simulink model "Fourteen_bus_simscape_V1o1"  (R2026a)
settings: Solver=ode23t  StopTime=12  FixedStep=0.2  RelTol=1e-2  AbsTol=1e-2  EnableMultiTasking=on
libraries: ee_lib x92, nesl_utility x64, fl_lib x25, eeRmsMeasurement x18, slpidlib x5, eeSmGovernor x2, elec_conv_HighZElecRef x1
(part 3 of 3)

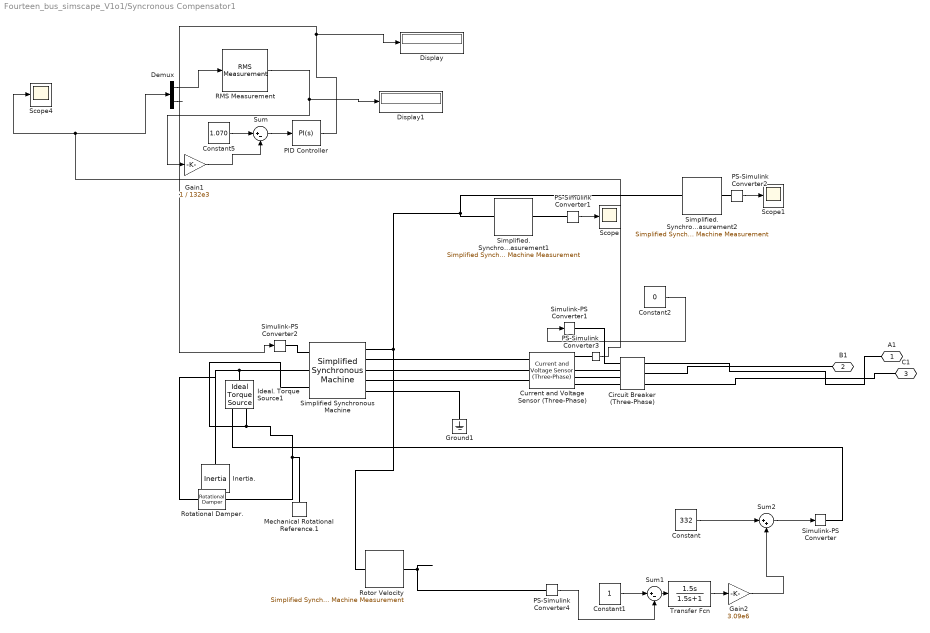
== system Fourteen_bus_simscape_V1o1/Syncronous Compensator1 ==
  Circuit Breaker (Three-Phase) : ee_lib/Switches & Breakers/Circuit Breaker (Three-Phase)  port_option=ee.enum.threePhasePort.expanded  control_port_option=ee.enum.controlport.ps  R_closed=0.001 Ohm  G_open=1e-6 1/Ohm  threshold=0.5 V  breaker_behavior=ee.enum.switches.breakerBehavior.zeroCrossingDisable  i_th=1e-8 A
  Constant : Constant  Value=332
  Constant1 : Constant
  Constant2 : Constant  Value=0
  Constant5 : Constant  Value=1.070
  Current and Voltage Sensor (Three-Phase) : ee_lib/Sensors & Transducers/Current and Voltage Sensor (Three-Phase)  port_option=ee.enum.threePhasePort.expanded  vMeasurementType=ee.enum.vmeasurement.ll  outputUnit=ee.enum.unit.si  SRated=100000000 V*A  VRated=0.95 V  I_specify=off  I_priority=None  I=[ 0 0 0 ] A  I_nominal_specify=off  I_nominal_value=1  I_nominal_unit=A  V_specify=off  V_priority=None  V=[ 0 0 0 ] V  V_nominal_specify=off  V_nominal_value=1  V_nominal_unit=V
  Demux : Demux  Outputs=3
  Display : Display
  Display1 : Display
  Gain1 : Gain  Gain=1 / 132e3
  Gain2 : Gain  Gain=3.09e6
  Ground1 : fl_lib/Electrical/Electrical Elements/Electrical Reference
  Ideal. Torque Source1 : fl_lib/Mechanical/Mechanical Sources/Ideal Torque Source
  Inertia. : fl_lib/Mechanical/Rotational Elements/Inertia  inertia=1.4e3 kg*m^2  num_ports=foundation.enum.numPorts2.one  w_specify=on  w_priority=High  w=377 rad/s  w_nominal_specify=off  w_nominal_value=1  w_nominal_unit=rad/s  t_specify=off  t_priority=None  t=0 N*m  t_nominal_specify=off  t_nominal_value=1  t_nominal_unit=N*m
  Mechanical Rotational Reference.1 : fl_lib/Mechanical/Rotational Elements/Mechanical Rotational Reference
  PID Controller : slpidlib/PID Controller  Controller=PI  Form=Parallel  TimeDomain=Continuous-time  UseExternalTs=off  SampleTime=-1  IntegratorMethod=Forward Euler  FilterMethod=Forward Euler  ControllerParametersSource=internal  P=1  I=10  UseKiTs=off  D=0  UseExternalDerivativeSource=off  N=100  UseFilter=on  TunerSelectOption=Transfer Function Based (PID Tuner App)  ZeroCross=off  InitialConditionSource=internal  InitialConditionForIntegrator=1  InitialConditionForFilter=0  DifferentiatorICPrevScaledInput=0  ExternalReset=none  TrackingMode=off  Kt=1  LimitOutput=on  SatLimitsSource=internal  UpperSaturationLimit=1.5  LowerSaturationLimit=0.5  LinearizeAsGain=on  AntiWindupMode=clamping  Kb=1  LimitIntegrator=off  UpperIntegratorSaturationLimit=inf  LowerIntegratorSaturationLimit=-inf  POutMin=[]  POutMax=[]  IOutMin=[]  IOutMax=[]  DOutMin=[]  DOutMax=[]  NOutMin=[]  NOutMax=[]  SumOutMin=[]  SumOutMax=[]  SaturationOutMin=[]  SaturationOutMax=[]  PParamMin=[]  PParamMax=[]  IParamMin=[]  IParamMax=[]  DParamMin=[]  DParamMax=[]  NParamMin=[]  NParamMax=[]  KbParamMin=[]  KbParamMax=[]  KtParamMin=[]  KtParamMax=[]  KbOutMin=[]  KbOutMax=[]  KtOutMin=[]  KtOutMax=[]  IntegratorOutMin=[]  IntegratorOutMax=[]  FilterOutMin=[]  FilterOutMax=[]  SumI1OutMin=[]  SumI1OutMax=[]  SumI2OutMin=[]  SumI2OutMax=[]  SumI3OutMin=[]  SumI3OutMax=[]  SumI4OutMin=[]  SumI4OutMax=[]  SumDOutMin=[]  SumDOutMax=[]  DifferentiatorOutMin=[]  DifferentiatorOutMax=[]  FilterDiffOutCoefMin=[]  FilterDiffOutCoefMax=[]  ReciprocalOutMin=[]  ReciprocalOutMax=[]  SumDenOutMin=[]  SumDenOutMax=[]  SumNumOutMin=[]  SumNumOutMax=[]  DivideOutMin=[]  DivideOutMax=[]  UdiffTsProdOutMin=[]  UdiffTsProdOutMax=[]  NTsProdOutMin=[]  NTsProdOutMax=[]  UintegralTsProdOutMin=[]  UintegralTsProdOutMax=[]  UngainTsProdOutMin=[]  UngainTsProdOutMax=[]  ClampingZeroOutDataTypeStr=Inherit: Inherit via back propagation  ClampingZeroOutMin=[]  ClampingZeroOutMax=[]  FilterDenConstantOutDataTypeStr=Inherit: Inherit via back propagation  FilterDenConstantOutMin=[]  FilterDenConstantOutMax=[]  PCopyOutDataTypeStr=Inherit: Inherit via back propagation  PCopyOutMin=[]  PCopyOutMax=[]  NCopyOutDataTypeStr=Inherit: Inherit via back propagation  NCopyOutMin=[]  NCopyOutMax=[]  IntegratorContinuousStateAttributes=''  IntegratorStateMustResolveToSignalObject=off  IntegratorRTWStateStorageClass=Auto  FilterContinuousStateAttributes=''  FilterStateMustResolveToSignalObject=off  FilterRTWStateStorageClass=Auto  ParallelPVariant=InternalParameters  IdealPVariant=Disabled  IVariant=InternalParameters  DVariant=Disabled  IntegratorVariant=Continuous  SatVariant=Enabled  AWVariant=ContClampingParallel  PCopyVariant=Disabled  TRVariant=Disabled  FdbkBlocksVariant=Forward  IdealPFdbkVariant=Disabled  SatFdbkVariant=Disabled  DerivativeFilterVariant=Disabled  NVariant=Disabled  NCopyVariant=Disabled_SignalSpec  FilterICVariant=Disabled  IntegratorICVariant=InternalICs  ExternalResetVariant=Disabled  TRSumVariant=Passthrough  SumFdbkVariant=Disabled  SumVariant=Sum_PI  TsampFilterVariant=InternalTs  TsampNgainVariant=Passthrough  TsampIntegralVariant=Disabled_SignalSpec  ExternalSaturationOutDataTypeStr=Inherit: Same as second input  DerivativeSourceVariant=Disabled  PreIntVariant=InternalPreInt
  PS-Simulink Converter{1..4} (4 alike) : nesl_utility/PS-Simulink Converter  PhysicalDomain=network_engine_domain  SubClassName=ps_output  LeftPortType=input  RightPortType=output  PseudoPeriodic=off  Frequencies=[]  VectorFormat=inherit  Unit=inherit  AffineConversion=off
  RMS Measurement : eeRmsMeasurement/RMS Measurement  LabelModeActiveChoice=Total  F=60  SpecifyHarmonics=off  K=[0 1 2]  Ts=0
      settings: LibrarySourceBlock=|
      | ee_sl_lib/Measurements/RMS
      | Measurement
  Rotational Damper. : fl_lib/Mechanical/Rotational Elements/Rotational Damper  D=0.88 N*m*s/rad  w_specify=off  w_priority=None  w=0 rad/s  w_nominal_specify=off  w_nominal_value=1  w_nominal_unit=rad/s  t_specify=off  t_priority=None  t=0 N*m  t_nominal_specify=off  t_nominal_value=1  t_nominal_unit=N*m
  Rotor Velocity : ee_lib/Electromechanical/Synchronous/Simplified Synchronous Machine Measurement  output_idx=5
  Scope : Scope
      settings: ActiveDisplayYMinimum=0.99179511268958387  ActiveDisplayYMaximum=1.0032727509539927  DataLoggingVariableName=ScopeData11
  Scope1 : Scope
      settings: ActiveDisplayYMinimum=-2.2503559561851616  ActiveDisplayYMaximum=3.0902333902320192  DataLoggingVariableName=ScopeData12
  Scope4 : Scope
      settings: ActiveDisplayYMinimum=-2.207198407413456E+9  ActiveDisplayYMaximum=1.6372196994728189E+9  DataLoggingVariableName=ScopeData13
  Simplified Synchronous Machine : ee_lib/Electromechanical/Synchronous/Simplified Synchronous Machine  port_option=ee.enum.threePhasePort.expanded  SRated=60e6 A*V  VRated=132e3 V  FRated=60 Hz  nPolePairs=1  param_unit=ee.enum.unit.pu  R_si=0.0519 Ohm  L_si=8.2589e-04 H  R_pu=0.0014  L_pu=0.232  initialization_option=ee.enum.sm.initialization.steadystate  source_type=ee.enum.sm.load_flow_source_type.PV  Vmag0=141240 V  Vang0=0 deg  Pt0=0 W  Qt0=0 A*V  minimum_pu=0.95  phase_search_range=[-inf, inf] deg  gmin=1e-6 S  connection_option=ee.enum.Connection.wye  angular_position_diff_specify=off  angular_position_diff_priority=None  angular_position_diff=0 rad  angular_position_diff_nominal_specify=off  angular_position_diff_nominal_value=1  angular_position_diff_nominal_unit=rad  pu_psid_specify=off  pu_psid_priority=None  pu_psid=0  pu_psid_nominal_specify=off  pu_psid_nominal_value=1  pu_psid_nominal_unit=1  pu_psiq_specify=off  pu_psiq_priority=None  pu_psiq=0  pu_psiq_nominal_specify=off  pu_psiq_nominal_value=1  pu_psiq_nominal_unit=1  pu_psi0_specify=off  pu_psi0_priority=None  pu_psi0=0  pu_psi0_nominal_specify=off  pu_psi0_nominal_value=1  pu_psi0_nominal_unit=1  angular_torque_specify=off  angular_torque_priority=None  angular_torque=0 N*m  angular_torque_nominal_specify=off  angular_torque_nominal_value=1  angular_torque_nominal_unit=N*m  Tmeas=298.15 K  alpha=3.93e-3 1/K  stator_thermal_mass=100 J/K  rotor_thermal_mass=200 J/K  temperatureA_specify=off  temperatureA_priority=High  temperatureA=25 degC  temperatureA_nominal_specify=off  temperatureA_nominal_value=1  temperatureA_nominal_unit=degC  temperatureB_specify=off  temperatureB_priority=High  temperatureB=25 degC  temperatureB_nominal_specify=off  temperatureB_nominal_value=1  temperatureB_nominal_unit=degC  temperatureC_specify=off  temperatureC_priority=High  temperatureC=25 degC  temperatureC_nominal_specify=off  temperatureC_nominal_value=1  temperatureC_nominal_unit=degC  temperatureR_specify=off  temperatureR_priority=High  temperatureR=25 degC  temperatureR_nominal_specify=off  temperatureR_nominal_value=1  temperatureR_nominal_unit=degC
  Simplified. Synchronous Machine Measurement1 : ee_lib/Electromechanical/Synchronous/Simplified Synchronous Machine Measurement  output_idx=5
  Simplified. Synchronous Machine Measurement2 : ee_lib/Electromechanical/Synchronous/Simplified Synchronous Machine Measurement  output_idx=4
  Simulink-PS Converter : nesl_utility/Simulink-PS Converter  PhysicalDomain=network_engine_domain  SubClassName=ps_input  LeftPortType=input  RightPortType=output  PseudoPeriodic=off  Frequencies=[]  NoiseDistribution=none  NoiseParameters=[]  Unit=1  AffineConversion=off  FilteringAndDerivatives=filter  SimscapeFilterOrder=1  InputFilterTimeConstant=0.001  UdotUserProvided=0
  Simulink-PS Converter1 : nesl_utility/Simulink-PS Converter  PhysicalDomain=network_engine_domain  SubClassName=ps_input  LeftPortType=input  RightPortType=output  PseudoPeriodic=off  Frequencies=[]  NoiseDistribution=none  NoiseParameters=[]  Unit=1  AffineConversion=off  FilteringAndDerivatives=provide  SimscapeFilterOrder=1  InputFilterTimeConstant=0.001  UdotUserProvided=0
  Simulink-PS Converter2 : nesl_utility/Simulink-PS Converter  PhysicalDomain=network_engine_domain  SubClassName=ps_input  LeftPortType=input  RightPortType=output  PseudoPeriodic=off  Frequencies=[]  NoiseDistribution=none  NoiseParameters=[]  Unit=1  AffineConversion=off  FilteringAndDerivatives=filter  SimscapeFilterOrder=1  InputFilterTimeConstant=0.001  UdotUserProvided=0
  Sum : Sum  Inputs=|+-
  Sum1 : Sum  Inputs=|+-
  Sum2 : Sum  Inputs=|++
  Transfer Fcn : TransferFcn  Numerator=[1.5 0]  Denominator=[1.5 1]
  A1 : PMIOPort  Side=Right
  B1 : PMIOPort  Port=2  Side=Right
  C1 : PMIOPort  Port=3  Side=Right
  wires:
  Constant1/1 -> Sum1/1
  PID Controller/1 -> Display/1, Simulink-PS Converter2/1
  Gain1/1 -> Sum/2
  Sum2/1 -> Simulink-PS Converter/1
  RMS Measurement/1 -> Display1/1, Gain1/1
  Transfer Fcn/1 -> Gain2/1
  Demux/1 -> RMS Measurement/1
  PS-Simulink Converter1/1 -> Scope/1
  PS-Simulink Converter2/1 -> Scope1/1
  Sum/1 -> PID Controller/1
  Constant/1 -> Sum2/1
  PS-Simulink Converter4/1 -> Sum1/2
  Demux/3 -> ?
  Gain2/1 -> Sum2/2
  Constant2/1 -> Simulink-PS Converter1/1
  Sum1/1 -> Transfer Fcn/1
  PS-Simulink Converter3/1 -> Demux/1, Scope4/1
  Constant5/1 -> Sum/1
  connections:
  Simplified Synchronous Machine/LConn2 -- Ideal. Torque Source1/LConn1 -- Inertia./LConn1 -- Rotational Damper./LConn1
  Rotor Velocity/RConn1 -- PS-Simulink Converter4/LConn1
  Mechanical Rotational Reference.1/LConn1 -- Rotational Damper./RConn1 -- Ideal. Torque Source1/RConn2 -- Simplified Synchronous Machine/LConn3
  Simplified. Synchronous Machine Measurement2/LConn1 -- Simplified. Synchronous Machine Measurement1/LConn1 -- Rotor Velocity/LConn1 -- Simplified Synchronous Machine/RConn1
  Circuit Breaker (Three-Phase)/RConn2 -- B1/RConn1
  Circuit Breaker (Three-Phase)/RConn1 -- A1/RConn1
  Simplified Synchronous Machine/LConn1 -- Simulink-PS Converter2/RConn1
  Simplified Synchronous Machine/RConn4 -- Current and Voltage Sensor (Three-Phase)/LConn3
  PS-Simulink Converter3/LConn1 -- Current and Voltage Sensor (Three-Phase)/RConn1
  Simplified Synchronous Machine/RConn3 -- Current and Voltage Sensor (Three-Phase)/LConn2
  Simplified Synchronous Machine/RConn5 -- Ground1/LConn1
  PS-Simulink Converter1/LConn1 -- Simplified. Synchronous Machine Measurement1/RConn1
  Simulink-PS Converter1/RConn1 -- Circuit Breaker (Three-Phase)/LConn1
  PS-Simulink Converter2/LConn1 -- Simplified. Synchronous Machine Measurement2/RConn1
  Circuit Breaker (Three-Phase)/LConn3 -- Current and Voltage Sensor (Three-Phase)/RConn4
  Simplified Synchronous Machine/RConn2 -- Current and Voltage Sensor (Three-Phase)/LConn1
  Circuit Breaker (Three-Phase)/LConn4 -- Current and Voltage Sensor (Three-Phase)/RConn5
  C1/RConn1 -- Circuit Breaker (Three-Phase)/RConn3
  Circuit Breaker (Three-Phase)/LConn2 -- Current and Voltage Sensor (Three-Phase)/RConn3
  Simulink-PS Converter/RConn1 -- Ideal. Torque Source1/RConn1

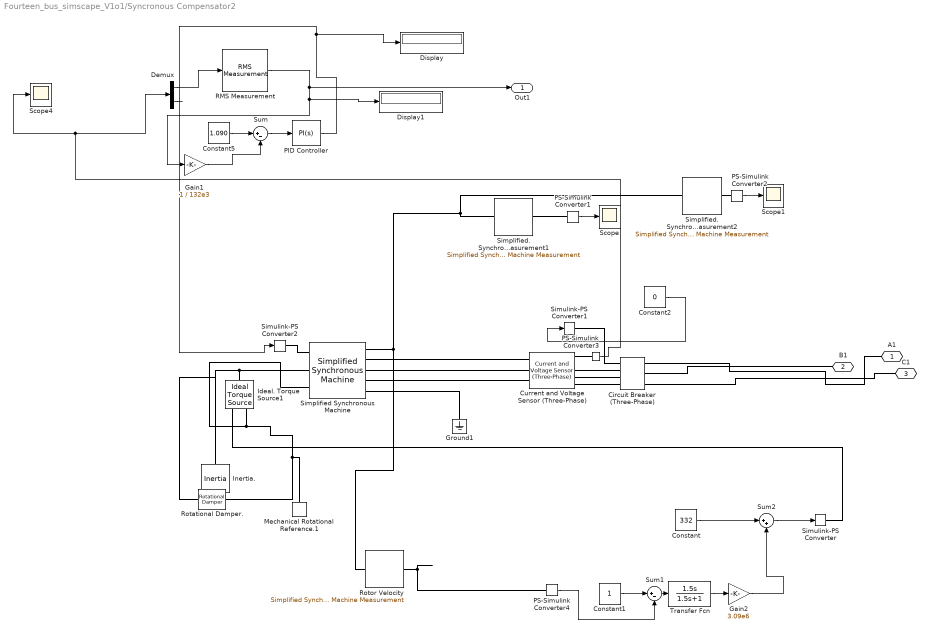
== system Fourteen_bus_simscape_V1o1/Syncronous Compensator2 ==
  Circuit Breaker (Three-Phase) : ee_lib/Switches & Breakers/Circuit Breaker (Three-Phase)  port_option=ee.enum.threePhasePort.expanded  control_port_option=ee.enum.controlport.ps  R_closed=0.001 Ohm  G_open=1e-6 1/Ohm  threshold=0.5 V  breaker_behavior=ee.enum.switches.breakerBehavior.zeroCrossingDisable  i_th=1e-8 A
  Constant : Constant  Value=332
  Constant1 : Constant
  Constant2 : Constant  Value=0
  Constant5 : Constant  Value=1.090
  Current and Voltage Sensor (Three-Phase) : ee_lib/Sensors & Transducers/Current and Voltage Sensor (Three-Phase)  port_option=ee.enum.threePhasePort.expanded  vMeasurementType=ee.enum.vmeasurement.ll  outputUnit=ee.enum.unit.si  SRated=100000000 V*A  VRated=0.95 V  I_specify=off  I_priority=None  I=[ 0 0 0 ] A  I_nominal_specify=off  I_nominal_value=1  I_nominal_unit=A  V_specify=off  V_priority=None  V=[ 0 0 0 ] V  V_nominal_specify=off  V_nominal_value=1  V_nominal_unit=V
  Demux : Demux  Outputs=3
  Display : Display
  Display1 : Display
  Gain1 : Gain  Gain=1 / 132e3
  Gain2 : Gain  Gain=3.09e6
  Ground1 : fl_lib/Electrical/Electrical Elements/Electrical Reference
  Ideal. Torque Source1 : fl_lib/Mechanical/Mechanical Sources/Ideal Torque Source
  Inertia. : fl_lib/Mechanical/Rotational Elements/Inertia  inertia=1.4e3 kg*m^2  num_ports=foundation.enum.numPorts2.one  w_specify=on  w_priority=High  w=377 rad/s  w_nominal_specify=off  w_nominal_value=1  w_nominal_unit=rad/s  t_specify=off  t_priority=None  t=0 N*m  t_nominal_specify=off  t_nominal_value=1  t_nominal_unit=N*m
  Mechanical Rotational Reference.1 : fl_lib/Mechanical/Rotational Elements/Mechanical Rotational Reference
  PID Controller : slpidlib/PID Controller  Controller=PI  Form=Parallel  TimeDomain=Continuous-time  UseExternalTs=off  SampleTime=-1  IntegratorMethod=Forward Euler  FilterMethod=Forward Euler  ControllerParametersSource=internal  P=1  I=10  UseKiTs=off  D=0  UseExternalDerivativeSource=off  N=100  UseFilter=on  TunerSelectOption=Transfer Function Based (PID Tuner App)  ZeroCross=off  InitialConditionSource=internal  InitialConditionForIntegrator=1  InitialConditionForFilter=0  DifferentiatorICPrevScaledInput=0  ExternalReset=none  TrackingMode=off  Kt=1  LimitOutput=on  SatLimitsSource=internal  UpperSaturationLimit=1.5  LowerSaturationLimit=0.5  LinearizeAsGain=on  AntiWindupMode=clamping  Kb=1  LimitIntegrator=off  UpperIntegratorSaturationLimit=inf  LowerIntegratorSaturationLimit=-inf  POutMin=[]  POutMax=[]  IOutMin=[]  IOutMax=[]  DOutMin=[]  DOutMax=[]  NOutMin=[]  NOutMax=[]  SumOutMin=[]  SumOutMax=[]  SaturationOutMin=[]  SaturationOutMax=[]  PParamMin=[]  PParamMax=[]  IParamMin=[]  IParamMax=[]  DParamMin=[]  DParamMax=[]  NParamMin=[]  NParamMax=[]  KbParamMin=[]  KbParamMax=[]  KtParamMin=[]  KtParamMax=[]  KbOutMin=[]  KbOutMax=[]  KtOutMin=[]  KtOutMax=[]  IntegratorOutMin=[]  IntegratorOutMax=[]  FilterOutMin=[]  FilterOutMax=[]  SumI1OutMin=[]  SumI1OutMax=[]  SumI2OutMin=[]  SumI2OutMax=[]  SumI3OutMin=[]  SumI3OutMax=[]  SumI4OutMin=[]  SumI4OutMax=[]  SumDOutMin=[]  SumDOutMax=[]  DifferentiatorOutMin=[]  DifferentiatorOutMax=[]  FilterDiffOutCoefMin=[]  FilterDiffOutCoefMax=[]  ReciprocalOutMin=[]  ReciprocalOutMax=[]  SumDenOutMin=[]  SumDenOutMax=[]  SumNumOutMin=[]  SumNumOutMax=[]  DivideOutMin=[]  DivideOutMax=[]  UdiffTsProdOutMin=[]  UdiffTsProdOutMax=[]  NTsProdOutMin=[]  NTsProdOutMax=[]  UintegralTsProdOutMin=[]  UintegralTsProdOutMax=[]  UngainTsProdOutMin=[]  UngainTsProdOutMax=[]  ClampingZeroOutDataTypeStr=Inherit: Inherit via back propagation  ClampingZeroOutMin=[]  ClampingZeroOutMax=[]  FilterDenConstantOutDataTypeStr=Inherit: Inherit via back propagation  FilterDenConstantOutMin=[]  FilterDenConstantOutMax=[]  PCopyOutDataTypeStr=Inherit: Inherit via back propagation  PCopyOutMin=[]  PCopyOutMax=[]  NCopyOutDataTypeStr=Inherit: Inherit via back propagation  NCopyOutMin=[]  NCopyOutMax=[]  IntegratorContinuousStateAttributes=''  IntegratorStateMustResolveToSignalObject=off  IntegratorRTWStateStorageClass=Auto  FilterContinuousStateAttributes=''  FilterStateMustResolveToSignalObject=off  FilterRTWStateStorageClass=Auto  ParallelPVariant=InternalParameters  IdealPVariant=Disabled  IVariant=InternalParameters  DVariant=Disabled  IntegratorVariant=Continuous  SatVariant=Enabled  AWVariant=ContClampingParallel  PCopyVariant=Disabled  TRVariant=Disabled  FdbkBlocksVariant=Forward  IdealPFdbkVariant=Disabled  SatFdbkVariant=Disabled  DerivativeFilterVariant=Disabled  NVariant=Disabled  NCopyVariant=Disabled_SignalSpec  FilterICVariant=Disabled  IntegratorICVariant=InternalICs  ExternalResetVariant=Disabled  TRSumVariant=Passthrough  SumFdbkVariant=Disabled  SumVariant=Sum_PI  TsampFilterVariant=InternalTs  TsampNgainVariant=Passthrough  TsampIntegralVariant=Disabled_SignalSpec  ExternalSaturationOutDataTypeStr=Inherit: Same as second input  DerivativeSourceVariant=Disabled  PreIntVariant=InternalPreInt
  PS-Simulink Converter{1..4} (4 alike) : nesl_utility/PS-Simulink Converter  PhysicalDomain=network_engine_domain  SubClassName=ps_output  LeftPortType=input  RightPortType=output  PseudoPeriodic=off  Frequencies=[]  VectorFormat=inherit  Unit=inherit  AffineConversion=off
  RMS Measurement : eeRmsMeasurement/RMS Measurement  LabelModeActiveChoice=Total  F=60  SpecifyHarmonics=off  K=[0 1 2]  Ts=0
      settings: LibrarySourceBlock=|
      | ee_sl_lib/Measurements/RMS
      | Measurement
  Rotational Damper. : fl_lib/Mechanical/Rotational Elements/Rotational Damper  D=0.88 N*m*s/rad  w_specify=off  w_priority=None  w=0 rad/s  w_nominal_specify=off  w_nominal_value=1  w_nominal_unit=rad/s  t_specify=off  t_priority=None  t=0 N*m  t_nominal_specify=off  t_nominal_value=1  t_nominal_unit=N*m
  Rotor Velocity : ee_lib/Electromechanical/Synchronous/Simplified Synchronous Machine Measurement  output_idx=5
  Scope : Scope
      settings: ActiveDisplayYMinimum=0.99105365347011376  ActiveDisplayYMaximum=1.0048917172693395  DataLoggingVariableName=ScopeData11
  Scope1 : Scope
      settings: ActiveDisplayYMinimum=-1.9277143555896115  ActiveDisplayYMaximum=4.9488574498751845  DataLoggingVariableName=ScopeData12
  Scope4 : Scope
      settings: ActiveDisplayYMinimum=-2.207198407413456E+9  ActiveDisplayYMaximum=1.6372196994728189E+9  DataLoggingVariableName=ScopeData13
  Simplified Synchronous Machine : ee_lib/Electromechanical/Synchronous/Simplified Synchronous Machine  port_option=ee.enum.threePhasePort.expanded  SRated=25e6 A*V  VRated=132e3 V  FRated=60 Hz  nPolePairs=1  param_unit=ee.enum.unit.pu  R_si=0.0519 Ohm  L_si=8.2589e-04 H  R_pu=0.0014  L_pu=0.232  initialization_option=ee.enum.sm.initialization.steadystate  source_type=ee.enum.sm.load_flow_source_type.PV  Vmag0=143880 V  Vang0=0 deg  Pt0=0 W  Qt0=0 A*V  minimum_pu=0.95  phase_search_range=[-inf, inf] deg  gmin=1e-6 S  connection_option=ee.enum.Connection.wye  angular_position_diff_specify=off  angular_position_diff_priority=None  angular_position_diff=0 rad  angular_position_diff_nominal_specify=off  angular_position_diff_nominal_value=1  angular_position_diff_nominal_unit=rad  pu_psid_specify=off  pu_psid_priority=None  pu_psid=0  pu_psid_nominal_specify=off  pu_psid_nominal_value=1  pu_psid_nominal_unit=1  pu_psiq_specify=off  pu_psiq_priority=None  pu_psiq=0  pu_psiq_nominal_specify=off  pu_psiq_nominal_value=1  pu_psiq_nominal_unit=1  pu_psi0_specify=off  pu_psi0_priority=None  pu_psi0=0  pu_psi0_nominal_specify=off  pu_psi0_nominal_value=1  pu_psi0_nominal_unit=1  angular_torque_specify=off  angular_torque_priority=None  angular_torque=0 N*m  angular_torque_nominal_specify=off  angular_torque_nominal_value=1  angular_torque_nominal_unit=N*m  Tmeas=298.15 K  alpha=3.93e-3 1/K  stator_thermal_mass=100 J/K  rotor_thermal_mass=200 J/K  temperatureA_specify=off  temperatureA_priority=High  temperatureA=25 degC  temperatureA_nominal_specify=off  temperatureA_nominal_value=1  temperatureA_nominal_unit=degC  temperatureB_specify=off  temperatureB_priority=High  temperatureB=25 degC  temperatureB_nominal_specify=off  temperatureB_nominal_value=1  temperatureB_nominal_unit=degC  temperatureC_specify=off  temperatureC_priority=High  temperatureC=25 degC  temperatureC_nominal_specify=off  temperatureC_nominal_value=1  temperatureC_nominal_unit=degC  temperatureR_specify=off  temperatureR_priority=High  temperatureR=25 degC  temperatureR_nominal_specify=off  temperatureR_nominal_value=1  temperatureR_nominal_unit=degC
  Simplified. Synchronous Machine Measurement1 : ee_lib/Electromechanical/Synchronous/Simplified Synchronous Machine Measurement  output_idx=5
  Simplified. Synchronous Machine Measurement2 : ee_lib/Electromechanical/Synchronous/Simplified Synchronous Machine Measurement  output_idx=4
  Simulink-PS Converter : nesl_utility/Simulink-PS Converter  PhysicalDomain=network_engine_domain  SubClassName=ps_input  LeftPortType=input  RightPortType=output  PseudoPeriodic=off  Frequencies=[]  NoiseDistribution=none  NoiseParameters=[]  Unit=1  AffineConversion=off  FilteringAndDerivatives=filter  SimscapeFilterOrder=1  InputFilterTimeConstant=0.001  UdotUserProvided=0
  Simulink-PS Converter1 : nesl_utility/Simulink-PS Converter  PhysicalDomain=network_engine_domain  SubClassName=ps_input  LeftPortType=input  RightPortType=output  PseudoPeriodic=off  Frequencies=[]  NoiseDistribution=none  NoiseParameters=[]  Unit=1  AffineConversion=off  FilteringAndDerivatives=provide  SimscapeFilterOrder=1  InputFilterTimeConstant=0.001  UdotUserProvided=0
  Simulink-PS Converter2 : nesl_utility/Simulink-PS Converter  PhysicalDomain=network_engine_domain  SubClassName=ps_input  LeftPortType=input  RightPortType=output  PseudoPeriodic=off  Frequencies=[]  NoiseDistribution=none  NoiseParameters=[]  Unit=1  AffineConversion=off  FilteringAndDerivatives=filter  SimscapeFilterOrder=1  InputFilterTimeConstant=0.001  UdotUserProvided=0
  Sum : Sum  Inputs=|+-
  Sum1 : Sum  Inputs=|+-
  Sum2 : Sum  Inputs=|++
  Transfer Fcn : TransferFcn  Numerator=[1.5 0]  Denominator=[1.5 1]
  A1 : PMIOPort  Side=Right
  B1 : PMIOPort  Port=2  Side=Right
  C1 : PMIOPort  Port=3  Side=Right
  Out1 : Outport
  wires:
  Constant1/1 -> Sum1/1
  PID Controller/1 -> Display/1, Simulink-PS Converter2/1
  Gain1/1 -> Sum/2
  Sum2/1 -> Simulink-PS Converter/1
  RMS Measurement/1 -> Out1/1, Display1/1, Gain1/1
  Transfer Fcn/1 -> Gain2/1
  Demux/1 -> RMS Measurement/1
  PS-Simulink Converter1/1 -> Scope/1
  PS-Simulink Converter2/1 -> Scope1/1
  Sum/1 -> PID Controller/1
  Constant/1 -> Sum2/1
  PS-Simulink Converter4/1 -> Sum1/2
  Demux/3 -> ?
  Gain2/1 -> Sum2/2
  Constant2/1 -> Simulink-PS Converter1/1
  Sum1/1 -> Transfer Fcn/1
  PS-Simulink Converter3/1 -> Demux/1, Scope4/1
  Constant5/1 -> Sum/1
  connections:
  Simplified Synchronous Machine/LConn2 -- Ideal. Torque Source1/LConn1 -- Inertia./LConn1 -- Rotational Damper./LConn1
  Rotor Velocity/RConn1 -- PS-Simulink Converter4/LConn1
  Mechanical Rotational Reference.1/LConn1 -- Rotational Damper./RConn1 -- Ideal. Torque Source1/RConn2 -- Simplified Synchronous Machine/LConn3
  Simplified. Synchronous Machine Measurement2/LConn1 -- Simplified. Synchronous Machine Measurement1/LConn1 -- Rotor Velocity/LConn1 -- Simplified Synchronous Machine/RConn1
  Circuit Breaker (Three-Phase)/RConn2 -- B1/RConn1
  Circuit Breaker (Three-Phase)/RConn1 -- A1/RConn1
  Simplified Synchronous Machine/LConn1 -- Simulink-PS Converter2/RConn1
  Simplified Synchronous Machine/RConn4 -- Current and Voltage Sensor (Three-Phase)/LConn3
  PS-Simulink Converter3/LConn1 -- Current and Voltage Sensor (Three-Phase)/RConn1
  Simplified Synchronous Machine/RConn3 -- Current and Voltage Sensor (Three-Phase)/LConn2
  Simplified Synchronous Machine/RConn5 -- Ground1/LConn1
  PS-Simulink Converter1/LConn1 -- Simplified. Synchronous Machine Measurement1/RConn1
  Simulink-PS Converter1/RConn1 -- Circuit Breaker (Three-Phase)/LConn1
  PS-Simulink Converter2/LConn1 -- Simplified. Synchronous Machine Measurement2/RConn1
  Circuit Breaker (Three-Phase)/LConn3 -- Current and Voltage Sensor (Three-Phase)/RConn4
  Simplified Synchronous Machine/RConn2 -- Current and Voltage Sensor (Three-Phase)/LConn1
  Circuit Breaker (Three-Phase)/LConn4 -- Current and Voltage Sensor (Three-Phase)/RConn5
  C1/RConn1 -- Circuit Breaker (Three-Phase)/RConn3
  Circuit Breaker (Three-Phase)/LConn2 -- Current and Voltage Sensor (Three-Phase)/RConn3
  Simulink-PS Converter/RConn1 -- Ideal. Torque Source1/RConn1

== system Fourteen_bus_simscape_V1o1/Three-Phase Series RL Branch2 ==
  Three_PhaseSeriesRLCBran : ee_lib/Passive/RLC Assemblies/RLC (Three-Phase)  port_option=ee.enum.threePhasePort.expanded  component_structure=ee.enum.rlc.structure.SeriesRL  R=3.377 Ohm  L=27.35 mH  C=1.471 uF  R_parasitic=1e-6 Ohm  G_parasitic=1e-6 1/Ohm  IL_specify=off  IL_priority=High  IL=[0, 0, 0] A  IL_nominal_specify=off  IL_nominal_value=1  IL_nominal_unit=A  VC_specify=off  VC_priority=High  VC=[0, 0, 0] V  VC_nominal_specify=off  VC_nominal_value=1  VC_nominal_unit=V
  A : PMIOPort  Side=Left
  B : PMIOPort  Port=2  Side=Left
  C : PMIOPort  Port=3  Side=Left
  a : PMIOPort  Port=4  Side=Right
  b : PMIOPort  Port=5  Side=Right
  c : PMIOPort  Port=6  Side=Right
  connections:
  Three_PhaseSeriesRLCBran/RConn3 -- c/RConn1
  Three_PhaseSeriesRLCBran/RConn2 -- b/RConn1
  Three_PhaseSeriesRLCBran/RConn1 -- a/RConn1
  C/RConn1 -- Three_PhaseSeriesRLCBran/LConn3
  B/RConn1 -- Three_PhaseSeriesRLCBran/LConn2
  A/RConn1 -- Three_PhaseSeriesRLCBran/LConn1

== system Fourteen_bus_simscape_V1o1/Three-Phase Series RLC Branch1 ==
  Three_PhaseSeriesRLCBran : ee_lib/Passive/RLC Assemblies/RLC (Three-Phase)  port_option=ee.enum.threePhasePort.expanded  component_structure=ee.enum.rlc.structure.SeriesRL  R=2.326 Ohm  L=19.46 mH  C=0.24868 F  R_parasitic=1e-6 Ohm  G_parasitic=1e-6 1/Ohm  IL_specify=off  IL_priority=High  IL=[0, 0, 0] A  IL_nominal_specify=off  IL_nominal_value=1  IL_nominal_unit=A  VC_specify=on  VC_priority=High  VC=[0, 0, 0] V  VC_nominal_specify=off  VC_nominal_value=1  VC_nominal_unit=V
  A : PMIOPort  Side=Left
  B : PMIOPort  Port=2  Side=Left
  C : PMIOPort  Port=3  Side=Left
  a : PMIOPort  Port=4  Side=Right
  b : PMIOPort  Port=5  Side=Right
  c : PMIOPort  Port=6  Side=Right
  connections:
  Three_PhaseSeriesRLCBran/RConn3 -- c/RConn1
  Three_PhaseSeriesRLCBran/RConn2 -- b/RConn1
  Three_PhaseSeriesRLCBran/RConn1 -- a/RConn1
  C/RConn1 -- Three_PhaseSeriesRLCBran/LConn3
  B/RConn1 -- Three_PhaseSeriesRLCBran/LConn2
  A/RConn1 -- Three_PhaseSeriesRLCBran/LConn1

== system Fourteen_bus_simscape_V1o1/Three-Phase Series RLC Branch10 ==
  Three_PhaseSeriesRLCBran : ee_lib/Passive/RLC Assemblies/RLC (Three-Phase)  port_option=ee.enum.threePhasePort.expanded  component_structure=2  R=1 Ohm  L=96.65 mH  C=1e-06 F  R_parasitic=1e-6 Ohm  G_parasitic=1e-6 1/Ohm  IL_specify=off  IL_priority=High  IL=[0, 0, 0] A  IL_nominal_specify=off  IL_nominal_value=1  IL_nominal_unit=A  VC_specify=on  VC_priority=High  VC=[0, 0, 0] V  VC_nominal_specify=off  VC_nominal_value=1  VC_nominal_unit=V
  B : PMIOPort  Side=Left
  A : PMIOPort  Port=2  Side=Left
  C : PMIOPort  Port=3  Side=Left
  a : PMIOPort  Port=4  Side=Right
  b : PMIOPort  Port=5  Side=Right
  c : PMIOPort  Port=6  Side=Right
  connections:
  Three_PhaseSeriesRLCBran/RConn3 -- c/RConn1
  Three_PhaseSeriesRLCBran/RConn2 -- b/RConn1
  Three_PhaseSeriesRLCBran/RConn1 -- a/RConn1
  C/RConn1 -- Three_PhaseSeriesRLCBran/LConn3
  B/RConn1 -- Three_PhaseSeriesRLCBran/LConn2
  A/RConn1 -- Three_PhaseSeriesRLCBran/LConn1

== system Fourteen_bus_simscape_V1o1/Three-Phase Series RLC Branch11 ==
  Three_PhaseSeriesRLCBran : ee_lib/Passive/RLC Assemblies/RLC (Three-Phase)  port_option=ee.enum.threePhasePort.expanded  component_structure=2  R=1 Ohm  L=50.85 mH  C=1e-06 F  R_parasitic=1e-6 Ohm  G_parasitic=1e-6 1/Ohm  IL_specify=off  IL_priority=High  IL=[0, 0, 0] A  IL_nominal_specify=off  IL_nominal_value=1  IL_nominal_unit=A  VC_specify=on  VC_priority=High  VC=[0, 0, 0] V  VC_nominal_specify=off  VC_nominal_value=1  VC_nominal_unit=V
  A : PMIOPort  Side=Left
  B : PMIOPort  Port=2  Side=Left
  C : PMIOPort  Port=3  Side=Left
  a : PMIOPort  Port=4  Side=Right
  b : PMIOPort  Port=5  Side=Right
  c : PMIOPort  Port=6  Side=Right
  connections:
  Three_PhaseSeriesRLCBran/RConn3 -- c/RConn1
  Three_PhaseSeriesRLCBran/RConn2 -- b/RConn1
  Three_PhaseSeriesRLCBran/RConn1 -- a/RConn1
  C/RConn1 -- Three_PhaseSeriesRLCBran/LConn3
  B/RConn1 -- Three_PhaseSeriesRLCBran/LConn2
  A/RConn1 -- Three_PhaseSeriesRLCBran/LConn1

== system Fourteen_bus_simscape_V1o1/Three-Phase Series RLC Branch12 ==
  Three_PhaseSeriesRLCBran : ee_lib/Passive/RLC Assemblies/RLC (Three-Phase)  port_option=ee.enum.threePhasePort.expanded  component_structure=4  R=16.550 Ohm  L=91.93 mH  C=1e-06 F  R_parasitic=1e-6 Ohm  G_parasitic=1e-6 1/Ohm  IL_specify=off  IL_priority=High  IL=[0, 0, 0] A  IL_nominal_specify=off  IL_nominal_value=1  IL_nominal_unit=A  VC_specify=on  VC_priority=High  VC=[0, 0, 0] V  VC_nominal_specify=off  VC_nominal_value=1  VC_nominal_unit=V
  A : PMIOPort  Side=Left
  B : PMIOPort  Port=2  Side=Left
  C : PMIOPort  Port=3  Side=Left
  a : PMIOPort  Port=4  Side=Right
  b : PMIOPort  Port=5  Side=Right
  c : PMIOPort  Port=6  Side=Right
  connections:
  Three_PhaseSeriesRLCBran/RConn3 -- c/RConn1
  Three_PhaseSeriesRLCBran/RConn2 -- b/RConn1
  Three_PhaseSeriesRLCBran/RConn1 -- a/RConn1
  C/RConn1 -- Three_PhaseSeriesRLCBran/LConn3
  B/RConn1 -- Three_PhaseSeriesRLCBran/LConn2
  A/RConn1 -- Three_PhaseSeriesRLCBran/LConn1

== system Fourteen_bus_simscape_V1o1/Three-Phase Series RLC Branch13 ==
  Three_PhaseSeriesRLCBran : ee_lib/Passive/RLC Assemblies/RLC (Three-Phase)  port_option=ee.enum.threePhasePort.expanded  component_structure=4  R=38.493 Ohm  L=92.38 mH  C=1e-06 F  R_parasitic=1e-6 Ohm  G_parasitic=1e-6 1/Ohm  IL_specify=off  IL_priority=High  IL=[0, 0, 0] A  IL_nominal_specify=off  IL_nominal_value=1  IL_nominal_unit=A  VC_specify=on  VC_priority=High  VC=[0, 0, 0] V  VC_nominal_specify=off  VC_nominal_value=1  VC_nominal_unit=V
  A : PMIOPort  Side=Left
  B : PMIOPort  Port=2  Side=Left
  C : PMIOPort  Port=3  Side=Left
  a : PMIOPort  Port=4  Side=Right
  b : PMIOPort  Port=5  Side=Right
  c : PMIOPort  Port=6  Side=Right
  connections:
  Three_PhaseSeriesRLCBran/RConn3 -- c/RConn1
  Three_PhaseSeriesRLCBran/RConn2 -- b/RConn1
  Three_PhaseSeriesRLCBran/RConn1 -- a/RConn1
  C/RConn1 -- Three_PhaseSeriesRLCBran/LConn3
  B/RConn1 -- Three_PhaseSeriesRLCBran/LConn2
  A/RConn1 -- Three_PhaseSeriesRLCBran/LConn1

== system Fourteen_bus_simscape_V1o1/Three-Phase Series RLC Branch14 ==
  Three_PhaseSeriesRLCBran : ee_lib/Passive/RLC Assemblies/RLC (Three-Phase)  port_option=ee.enum.threePhasePort.expanded  component_structure=4  R=29.783 Ohm  L=160.85 mH  C=1e-06 F  R_parasitic=1e-6 Ohm  G_parasitic=1e-6 1/Ohm  IL_specify=off  IL_priority=High  IL=[0, 0, 0] A  IL_nominal_specify=off  IL_nominal_value=1  IL_nominal_unit=A  VC_specify=on  VC_priority=High  VC=[0, 0, 0] V  VC_nominal_specify=off  VC_nominal_value=1  VC_nominal_unit=V
  A : PMIOPort  Side=Left
  B : PMIOPort  Port=2  Side=Left
  C : PMIOPort  Port=3  Side=Left
  a : PMIOPort  Port=4  Side=Right
  b : PMIOPort  Port=5  Side=Right
  c : PMIOPort  Port=6  Side=Right
  connections:
  Three_PhaseSeriesRLCBran/RConn3 -- c/RConn1
  Three_PhaseSeriesRLCBran/RConn2 -- b/RConn1
  Three_PhaseSeriesRLCBran/RConn1 -- a/RConn1
  C/RConn1 -- Three_PhaseSeriesRLCBran/LConn3
  B/RConn1 -- Three_PhaseSeriesRLCBran/LConn2
  A/RConn1 -- Three_PhaseSeriesRLCBran/LConn1

== system Fourteen_bus_simscape_V1o1/Three-Phase Series RLC Branch15 ==
  Three_PhaseSeriesRLCBran : ee_lib/Passive/RLC Assemblies/RLC (Three-Phase)  port_option=ee.enum.threePhasePort.expanded  component_structure=4  R=21.420 Ohm  L=118.23 mH  C=1e-06 F  R_parasitic=1e-6 Ohm  G_parasitic=1e-6 1/Ohm  IL_specify=off  IL_priority=High  IL=[0, 0, 0] A  IL_nominal_specify=off  IL_nominal_value=1  IL_nominal_unit=A  VC_specify=on  VC_priority=High  VC=[0, 0, 0] V  VC_nominal_specify=off  VC_nominal_value=1  VC_nominal_unit=V
  A : PMIOPort  Side=Left
  B : PMIOPort  Port=2  Side=Left
  C : PMIOPort  Port=3  Side=Left
  a : PMIOPort  Port=4  Side=Right
  b : PMIOPort  Port=5  Side=Right
  c : PMIOPort  Port=6  Side=Right
  connections:
  Three_PhaseSeriesRLCBran/RConn3 -- c/RConn1
  Three_PhaseSeriesRLCBran/RConn2 -- b/RConn1
  Three_PhaseSeriesRLCBran/RConn1 -- a/RConn1
  C/RConn1 -- Three_PhaseSeriesRLCBran/LConn3
  B/RConn1 -- Three_PhaseSeriesRLCBran/LConn2
  A/RConn1 -- Three_PhaseSeriesRLCBran/LConn1

== system Fourteen_bus_simscape_V1o1/Three-Phase Series RLC Branch16 ==
  Three_PhaseSeriesRLCBran : ee_lib/Passive/RLC Assemblies/RLC (Three-Phase)  port_option=ee.enum.threePhasePort.expanded  component_structure=4  R=22.148 Ohm  L=124.97 mH  C=1e-06 F  R_parasitic=1e-6 Ohm  G_parasitic=1e-6 1/Ohm  IL_specify=off  IL_priority=High  IL=[0, 0, 0] A  IL_nominal_specify=off  IL_nominal_value=1  IL_nominal_unit=A  VC_specify=on  VC_priority=High  VC=[0, 0, 0] V  VC_nominal_specify=off  VC_nominal_value=1  VC_nominal_unit=V
  A : PMIOPort  Side=Left
  B : PMIOPort  Port=2  Side=Left
  C : PMIOPort  Port=3  Side=Left
  a : PMIOPort  Port=4  Side=Right
  b : PMIOPort  Port=5  Side=Right
  c : PMIOPort  Port=6  Side=Right
  connections:
  Three_PhaseSeriesRLCBran/RConn3 -- c/RConn1
  Three_PhaseSeriesRLCBran/RConn2 -- b/RConn1
  Three_PhaseSeriesRLCBran/RConn1 -- a/RConn1
  C/RConn1 -- Three_PhaseSeriesRLCBran/LConn3
  B/RConn1 -- Three_PhaseSeriesRLCBran/LConn2
  A/RConn1 -- Three_PhaseSeriesRLCBran/LConn1

== system Fourteen_bus_simscape_V1o1/Three-Phase Series RLC Branch17 ==
  Three_PhaseSeriesRLCBran : ee_lib/Passive/RLC Assemblies/RLC (Three-Phase)  port_option=ee.enum.threePhasePort.expanded  component_structure=4  R=5.543 Ohm  L=39.06 mH  C=1e-06 F  R_parasitic=1e-6 Ohm  G_parasitic=1e-6 1/Ohm  IL_specify=off  IL_priority=High  IL=[0, 0, 0] A  IL_nominal_specify=off  IL_nominal_value=1  IL_nominal_unit=A  VC_specify=on  VC_priority=High  VC=[0, 0, 0] V  VC_nominal_specify=off  VC_nominal_value=1  VC_nominal_unit=V
  A : PMIOPort  Side=Left
  B : PMIOPort  Port=2  Side=Left
  C : PMIOPort  Port=3  Side=Left
  a : PMIOPort  Port=4  Side=Right
  b : PMIOPort  Port=5  Side=Right
  c : PMIOPort  Port=6  Side=Right
  connections:
  Three_PhaseSeriesRLCBran/RConn3 -- c/RConn1
  Three_PhaseSeriesRLCBran/RConn2 -- b/RConn1
  Three_PhaseSeriesRLCBran/RConn1 -- a/RConn1
  C/RConn1 -- Three_PhaseSeriesRLCBran/LConn3
  B/RConn1 -- Three_PhaseSeriesRLCBran/LConn2
  A/RConn1 -- Three_PhaseSeriesRLCBran/LConn1

== system Fourteen_bus_simscape_V1o1/Three-Phase Series RLC Branch18 ==
  Three_PhaseSeriesRLCBran : ee_lib/Passive/RLC Assemblies/RLC (Three-Phase)  port_option=ee.enum.threePhasePort.expanded  component_structure=4  R=11.530 Ohm  L=60.21 mH  C=1e-06 F  R_parasitic=1e-6 Ohm  G_parasitic=1e-6 1/Ohm  IL_specify=off  IL_priority=High  IL=[0, 0, 0] A  IL_nominal_specify=off  IL_nominal_value=1  IL_nominal_unit=A  VC_specify=on  VC_priority=High  VC=[0, 0, 0] V  VC_nominal_specify=off  VC_nominal_value=1  VC_nominal_unit=V
  A : PMIOPort  Side=Left
  B : PMIOPort  Port=2  Side=Left
  C : PMIOPort  Port=3  Side=Left
  a : PMIOPort  Port=4  Side=Right
  b : PMIOPort  Port=5  Side=Right
  c : PMIOPort  Port=6  Side=Right
  connections:
  Three_PhaseSeriesRLCBran/RConn3 -- c/RConn1
  Three_PhaseSeriesRLCBran/RConn2 -- b/RConn1
  Three_PhaseSeriesRLCBran/RConn1 -- a/RConn1
  C/RConn1 -- Three_PhaseSeriesRLCBran/LConn3
  B/RConn1 -- Three_PhaseSeriesRLCBran/LConn2
  A/RConn1 -- Three_PhaseSeriesRLCBran/LConn1

== system Fourteen_bus_simscape_V1o1/Three-Phase Series RLC Branch19 ==
  Three_PhaseSeriesRLCBran : ee_lib/Passive/RLC Assemblies/RLC (Three-Phase)  port_option=ee.enum.threePhasePort.expanded  component_structure=4  R=14.296 Ohm  L=88.77 mH  C=1e-06 F  R_parasitic=1e-6 Ohm  G_parasitic=1e-6 1/Ohm  IL_specify=off  IL_priority=High  IL=[0, 0, 0] A  IL_nominal_specify=off  IL_nominal_value=1  IL_nominal_unit=A  VC_specify=on  VC_priority=High  VC=[0, 0, 0] V  VC_nominal_specify=off  VC_nominal_value=1  VC_nominal_unit=V
  A : PMIOPort  Side=Left
  B : PMIOPort  Port=2  Side=Left
  C : PMIOPort  Port=3  Side=Left
  a : PMIOPort  Port=4  Side=Right
  b : PMIOPort  Port=5  Side=Right
  c : PMIOPort  Port=6  Side=Right
  connections:
  Three_PhaseSeriesRLCBran/RConn3 -- c/RConn1
  Three_PhaseSeriesRLCBran/RConn2 -- b/RConn1
  Three_PhaseSeriesRLCBran/RConn1 -- a/RConn1
  C/RConn1 -- Three_PhaseSeriesRLCBran/LConn3
  B/RConn1 -- Three_PhaseSeriesRLCBran/LConn2
  A/RConn1 -- Three_PhaseSeriesRLCBran/LConn1

== system Fourteen_bus_simscape_V1o1/Three-Phase Series RLC Branch20 ==
  Three_PhaseSeriesRLCBran : ee_lib/Passive/RLC Assemblies/RLC (Three-Phase)  port_option=ee.enum.threePhasePort.expanded  component_structure=ee.enum.rlc.structure.SeriesRL  R=9.923 Ohm  L=80.37 mH  C=0.964 uF  R_parasitic=1e-6 Ohm  G_parasitic=1e-6 1/Ohm  IL_specify=off  IL_priority=High  IL=[0, 0, 0] A  IL_nominal_specify=off  IL_nominal_value=1  IL_nominal_unit=A  VC_specify=off  VC_priority=High  VC=[0, 0, 0] V  VC_nominal_specify=off  VC_nominal_value=1  VC_nominal_unit=V
  A : PMIOPort  Side=Left
  B : PMIOPort  Port=2  Side=Left
  C : PMIOPort  Port=3  Side=Left
  a : PMIOPort  Port=4  Side=Right
  b : PMIOPort  Port=5  Side=Right
  c : PMIOPort  Port=6  Side=Right
  connections:
  Three_PhaseSeriesRLCBran/RConn3 -- c/RConn1
  Three_PhaseSeriesRLCBran/RConn2 -- b/RConn1
  Three_PhaseSeriesRLCBran/RConn1 -- a/RConn1
  C/RConn1 -- Three_PhaseSeriesRLCBran/LConn3
  B/RConn1 -- Three_PhaseSeriesRLCBran/LConn2
  A/RConn1 -- Three_PhaseSeriesRLCBran/LConn1

== system Fourteen_bus_simscape_V1o1/Three-Phase Series RLC Branch3 ==
  Three_PhaseSeriesRLCBran : ee_lib/Passive/RLC Assemblies/RLC (Three-Phase)  port_option=ee.enum.threePhasePort.expanded  component_structure=ee.enum.rlc.structure.SeriesRL  R=8.187 Ohm  L=91.50 mH  C=1.220 uF  R_parasitic=1e-6 Ohm  G_parasitic=1e-6 1/Ohm  IL_specify=off  IL_priority=High  IL=[0, 0, 0] A  IL_nominal_specify=off  IL_nominal_value=1  IL_nominal_unit=A  VC_specify=off  VC_priority=High  VC=[0, 0, 0] V  VC_nominal_specify=off  VC_nominal_value=1  VC_nominal_unit=V
  A : PMIOPort  Side=Left
  B : PMIOPort  Port=2  Side=Left
  C : PMIOPort  Port=3  Side=Left
  a : PMIOPort  Port=4  Side=Right
  b : PMIOPort  Port=5  Side=Right
  c : PMIOPort  Port=6  Side=Right
  connections:
  Three_PhaseSeriesRLCBran/RConn3 -- c/RConn1
  Three_PhaseSeriesRLCBran/RConn2 -- b/RConn1
  Three_PhaseSeriesRLCBran/RConn1 -- a/RConn1
  C/RConn1 -- Three_PhaseSeriesRLCBran/LConn3
  B/RConn1 -- Three_PhaseSeriesRLCBran/LConn2
  A/RConn1 -- Three_PhaseSeriesRLCBran/LConn1

== system Fourteen_bus_simscape_V1o1/Three-Phase Series RLC Branch4 ==
  Three_PhaseSeriesRLCBran : ee_lib/Passive/RLC Assemblies/RLC (Three-Phase)  port_option=ee.enum.threePhasePort.expanded  component_structure=2  R=1 Ohm  L=116.48 mH  C=1e-06 F  R_parasitic=1e-6 Ohm  G_parasitic=1e-6 1/Ohm  IL_specify=off  IL_priority=High  IL=[0, 0, 0] A  IL_nominal_specify=off  IL_nominal_value=1  IL_nominal_unit=A  VC_specify=on  VC_priority=High  VC=[0, 0, 0] V  VC_nominal_specify=off  VC_nominal_value=1  VC_nominal_unit=V
  A : PMIOPort  Side=Left
  B : PMIOPort  Port=2  Side=Left
  C : PMIOPort  Port=3  Side=Left
  a : PMIOPort  Port=4  Side=Right
  b : PMIOPort  Port=5  Side=Right
  c : PMIOPort  Port=6  Side=Right
  connections:
  Three_PhaseSeriesRLCBran/RConn3 -- c/RConn1
  Three_PhaseSeriesRLCBran/RConn2 -- b/RConn1
  Three_PhaseSeriesRLCBran/RConn1 -- a/RConn1
  C/RConn1 -- Three_PhaseSeriesRLCBran/LConn3
  B/RConn1 -- Three_PhaseSeriesRLCBran/LConn2
  A/RConn1 -- Three_PhaseSeriesRLCBran/LConn1

== system Fourteen_bus_simscape_V1o1/Three-Phase Series RLC Branch5 ==
  Three_PhaseSeriesRLCBran : ee_lib/Passive/RLC Assemblies/RLC (Three-Phase)  port_option=ee.enum.threePhasePort.expanded  component_structure=ee.enum.rlc.structure.SeriesRL  R=11.676 Ohm  L=79.05 mH  C=0.357 F  R_parasitic=1e-6 Ohm  G_parasitic=1e-6 1/Ohm  IL_specify=off  IL_priority=High  IL=[0, 0, 0] A  IL_nominal_specify=off  IL_nominal_value=1  IL_nominal_unit=A  VC_specify=off  VC_priority=High  VC=[0, 0, 0] V  VC_nominal_specify=off  VC_nominal_value=1  VC_nominal_unit=V
  A : PMIOPort  Side=Left
  B : PMIOPort  Port=2  Side=Left
  C : PMIOPort  Port=3  Side=Left
  a : PMIOPort  Port=4  Side=Right
  b : PMIOPort  Port=5  Side=Right
  c : PMIOPort  Port=6  Side=Right
  connections:
  Three_PhaseSeriesRLCBran/RConn3 -- c/RConn1
  Three_PhaseSeriesRLCBran/RConn2 -- b/RConn1
  Three_PhaseSeriesRLCBran/RConn1 -- a/RConn1
  C/RConn1 -- Three_PhaseSeriesRLCBran/LConn3
  B/RConn1 -- Three_PhaseSeriesRLCBran/LConn2
  A/RConn1 -- Three_PhaseSeriesRLCBran/LConn1

== system Fourteen_bus_simscape_V1o1/Three-Phase Series RLC Branch6 ==
  Three_PhaseSeriesRLCBran : ee_lib/Passive/RLC Assemblies/RLC (Three-Phase)  port_option=ee.enum.threePhasePort.expanded  component_structure=ee.enum.rlc.structure.SeriesRL  R=10.125 Ohm  L=81.50 mH  C=0.947 uF  R_parasitic=1e-6 Ohm  G_parasitic=1e-6 1/Ohm  IL_specify=off  IL_priority=High  IL=[0, 0, 0] A  IL_nominal_specify=off  IL_nominal_value=1  IL_nominal_unit=A  VC_specify=off  VC_priority=High  VC=[0, 0, 0] V  VC_nominal_specify=off  VC_nominal_value=1  VC_nominal_unit=V
  A : PMIOPort  Side=Left
  B : PMIOPort  Port=2  Side=Left
  C : PMIOPort  Port=3  Side=Left
  a : PMIOPort  Port=4  Side=Right
  b : PMIOPort  Port=5  Side=Right
  c : PMIOPort  Port=6  Side=Right
  connections:
  Three_PhaseSeriesRLCBran/RConn3 -- c/RConn1
  Three_PhaseSeriesRLCBran/RConn2 -- b/RConn1
  Three_PhaseSeriesRLCBran/RConn1 -- a/RConn1
  C/RConn1 -- Three_PhaseSeriesRLCBran/LConn3
  B/RConn1 -- Three_PhaseSeriesRLCBran/LConn2
  A/RConn1 -- Three_PhaseSeriesRLCBran/LConn1

== system Fourteen_bus_simscape_V1o1/Three-Phase Series RLC Branch7 ==
  Three_PhaseSeriesRLCBran : ee_lib/Passive/RLC Assemblies/RLC (Three-Phase)  port_option=ee.enum.threePhasePort.expanded  component_structure=ee.enum.rlc.structure.SeriesRL  R=9.414 Ohm  L=103.10 mH  C=1.371 uF  R_parasitic=1e-6 Ohm  G_parasitic=1e-6 1/Ohm  IL_specify=off  IL_priority=High  IL=[0, 0, 0] A  IL_nominal_specify=off  IL_nominal_value=1  IL_nominal_unit=A  VC_specify=off  VC_priority=High  VC=[0, 0, 0] V  VC_nominal_specify=off  VC_nominal_value=1  VC_nominal_unit=V
  A : PMIOPort  Side=Left
  B : PMIOPort  Port=2  Side=Left
  C : PMIOPort  Port=3  Side=Left
  a : PMIOPort  Port=4  Side=Right
  b : PMIOPort  Port=5  Side=Right
  c : PMIOPort  Port=6  Side=Right
  connections:
  Three_PhaseSeriesRLCBran/RConn3 -- c/RConn1
  Three_PhaseSeriesRLCBran/RConn2 -- b/RConn1
  Three_PhaseSeriesRLCBran/RConn1 -- a/RConn1
  C/RConn1 -- Three_PhaseSeriesRLCBran/LConn3
  B/RConn1 -- Three_PhaseSeriesRLCBran/LConn2
  A/RConn1 -- Three_PhaseSeriesRLCBran/LConn1

== system Fourteen_bus_simscape_V1o1/Three-Phase Series RLC Branch8 ==
  Three_PhaseSeriesRLCBran : ee_lib/Passive/RLC Assemblies/RLC (Three-Phase)  port_option=ee.enum.threePhasePort.expanded  component_structure=2  R=1 Ohm  L=257.06 mH  C=1e-06 F  R_parasitic=1e-6 Ohm  G_parasitic=1e-6 1/Ohm  IL_specify=off  IL_priority=High  IL=[0, 0, 0] A  IL_nominal_specify=off  IL_nominal_value=1  IL_nominal_unit=A  VC_specify=on  VC_priority=High  VC=[0, 0, 0] V  VC_nominal_specify=off  VC_nominal_value=1  VC_nominal_unit=V
  A : PMIOPort  Side=Left
  B : PMIOPort  Port=2  Side=Left
  C : PMIOPort  Port=3  Side=Left
  a : PMIOPort  Port=4  Side=Right
  b : PMIOPort  Port=5  Side=Right
  c : PMIOPort  Port=6  Side=Right
  connections:
  Three_PhaseSeriesRLCBran/RConn3 -- c/RConn1
  Three_PhaseSeriesRLCBran/RConn2 -- b/RConn1
  Three_PhaseSeriesRLCBran/RConn1 -- a/RConn1
  C/RConn1 -- Three_PhaseSeriesRLCBran/LConn3
  B/RConn1 -- Three_PhaseSeriesRLCBran/LConn2
  A/RConn1 -- Three_PhaseSeriesRLCBran/LConn1

== system Fourteen_bus_simscape_V1o1/Three-Phase Series RLC Branch9 ==
  Three_PhaseSeriesRLCBran : ee_lib/Passive/RLC Assemblies/RLC (Three-Phase)  port_option=ee.enum.threePhasePort.expanded  component_structure=2  R=1 Ohm  L=81.41 mH  C=1e-06 F  R_parasitic=1e-6 Ohm  G_parasitic=1e-6 1/Ohm  IL_specify=on  IL_priority=High  IL=[0, 0, 0] A  IL_nominal_specify=off  IL_nominal_value=1  IL_nominal_unit=A  VC_specify=on  VC_priority=High  VC=[0, 0, 0] V  VC_nominal_specify=off  VC_nominal_value=1  VC_nominal_unit=V
  A : PMIOPort  Side=Left
  B : PMIOPort  Port=2  Side=Left
  C : PMIOPort  Port=3  Side=Left
  a : PMIOPort  Port=4  Side=Right
  b : PMIOPort  Port=5  Side=Right
  c : PMIOPort  Port=6  Side=Right
  connections:
  Three_PhaseSeriesRLCBran/RConn3 -- c/RConn1
  Three_PhaseSeriesRLCBran/RConn2 -- b/RConn1
  Three_PhaseSeriesRLCBran/RConn1 -- a/RConn1
  C/RConn1 -- Three_PhaseSeriesRLCBran/LConn3
  B/RConn1 -- Three_PhaseSeriesRLCBran/LConn2
  A/RConn1 -- Three_PhaseSeriesRLCBran/LConn1
